simulink model "fw_implement_aux"  (R2026b)
settings: Solver=VariableStepAuto
undefined symbols (not defined in the file or in its folder): ImplementType, P, ShaddadMode, Ts
libraries: simulink x38
settings Model: Creator=aomar  LastModifiedBy=aomar

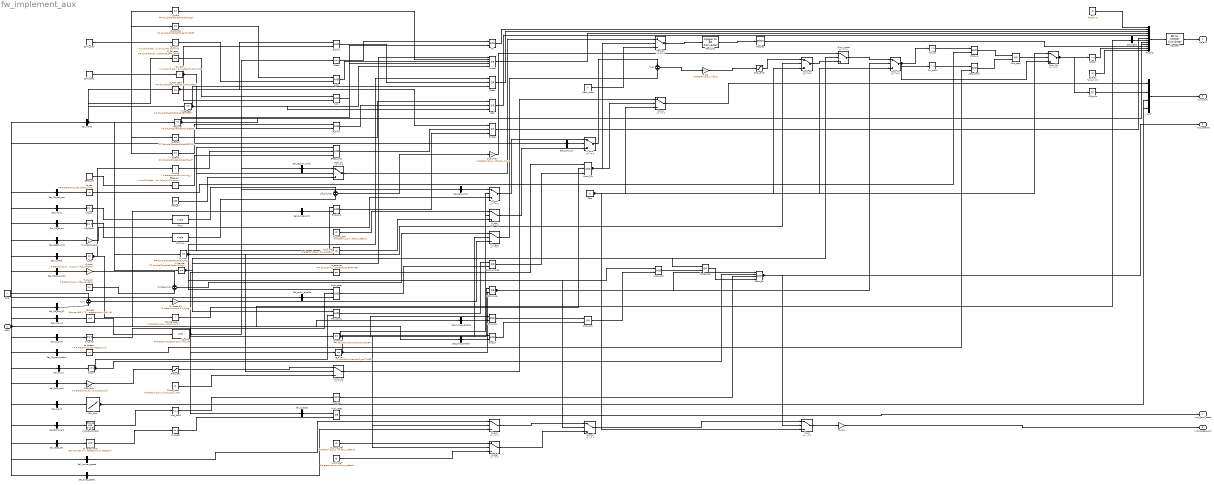
== system fw_implement_aux ==
  fw50 : Inport  SampleTime=Ts.comm
  A_cs : Logic  AllPortsSameDT=off  OutDataTypeStr=boolean
  A_sb : Logic  AllPortsSameDT=off  OutDataTypeStr=boolean
  Amber : Logic  Operator=OR  Inputs=5  AllPortsSameDT=off  OutDataTypeStr=boolean
  At_bottom : simulink/Logic and Bit Operations/Compare To Constant  relop=<=  const=P.electronics.adc.liftpot_lim(1)  OutDataTypeStr=boolean
  At_top : simulink/Logic and Bit Operations/Compare To Constant  relop=>=  const=P.electronics.adc.liftpot_lim(2)  OutDataTypeStr=boolean
  Auto_rotor : Logic  AllPortsSameDT=off  OutDataTypeStr=boolean
  Auto_spray : Logic  Inputs=3  AllPortsSameDT=off  OutDataTypeStr=boolean
  B01 : Constant  Value=false(1,2)  OutDataTypeStr=boolean  SampleTime=Ts.comm
  B19_31 : Constant  Value=false(1,13)  OutDataTypeStr=boolean  SampleTime=Ts.comm
  Beep_auto : Logic  Inputs=3  AllPortsSameDT=off  OutDataTypeStr=boolean
  Beep_cnt : simulink/Sources/Counter Limited  uplimit=round(P.electronics.aux.buzz_period/Ts.comm) - 1  tsamp=Ts.comm
  Beep_on : simulink/Logic and Bit Operations/Compare To Constant  relop=<  const=round(P.electronics.aux.buzz_on/Ts.comm)  OutDataTypeStr=boolean
  Blink_fast : simulink/Sources/Counter Limited  uplimit=round(1/(P.electronics.aux.blink_fast*Ts.comm)) - 1  tsamp=Ts.comm
  Blink_slow : simulink/Sources/Counter Limited  uplimit=round(1/(P.electronics.aux.blink_f*Ts.comm)) - 1  tsamp=Ts.comm
  Buzzer : Logic  Operator=OR  Inputs=3  AllPortsSameDT=off  OutDataTypeStr=boolean
  Di_reset : simulink/Logic and Bit Operations/Compare To Zero  relop=~=  OutDataTypeStr=boolean
  Di_reset_mask : simulink/Logic and Bit Operations/Bitwise Operator  logicop=AND  UseBitMask=on  BitMask=2^(P.electronics.di.reset_btn)  BitMaskRealWorld=Stored Integer
  Dir_down : simulink/Logic and Bit Operations/Compare To Zero  relop=<  OutDataTypeStr=boolean
  Dir_up : simulink/Logic and Bit Operations/Compare To Zero  relop=>  OutDataTypeStr=boolean
  Do_bits : Concatenate  NumInputs=12
  Do_pack : simulink/Logic and Bit Operations/Bit to Integer Converter  nbits=32  bitOrder=LSB first  signedOutputValues=Unsigned  outDtype=uint32  outDtypeSigned=Inherit via internal rule
      settings: LibrarySourceBlock=|
      | commutil2/Bit to Integer
      | Converter
  Down_s : DataTypeConversion  OutDataTypeStr=single  RndMeth=Round
  Duty_a0 : Switch  Criteria=u2 ~= 0  SaturateOnIntegerOverflow=off  InputSameDT=off
  Duty_auto : Saturate  UpperLimit=P.electronics.aux.lift_duty_max  LowerLimit=-P.electronics.aux.lift_duty_max
  Duty_fit : Switch  Criteria=u2 ~= 0  SaturateOnIntegerOverflow=off  InputSameDT=off
  Duty_lift : Switch  Criteria=u2 ~= 0  SaturateOnIntegerOverflow=off  InputSameDT=off
  Duty_man : Gain  Gain=P.electronics.aux.lift_duty_max
  Duty_mode : Switch  Criteria=u2 ~= 0  SaturateOnIntegerOverflow=off  InputSameDT=off
  End_stop : Logic  Operator=OR  AllPortsSameDT=off  OutDataTypeStr=boolean
  Fan_duty : Lookup_n-D  NumberOfTableDimensions=1  BreakpointsForDimension1=P.electronics.aux.fan_bp  BreakpointsForDimension1DataTypeStr=single  Table=P.electronics.aux.fan_duty  TableDataTypeStr=single  ExtrapMethod=Clip  InternalRulePriority=Speed  OutDataTypeStr=single  RndMeth=Simplest
  Fitted : simulink/Logic and Bit Operations/Compare To Constant  relop=~=  const=0  OutDataTypeStr=boolean
  Flow_duty : Gain  Gain=1/P.electronics.aux.pump_flow_full
  Flow_sat : Saturate  UpperLimit=1  LowerLimit=0
  G_blink : Logic  AllPortsSameDT=off  OutDataTypeStr=boolean
  Gnc_buzz : Logic  AllPortsSameDT=off  OutDataTypeStr=boolean
  Gnc_mow : Logic  AllPortsSameDT=off  OutDataTypeStr=boolean
  Gnc_rotor : Logic  Operator=OR  AllPortsSameDT=off  OutDataTypeStr=boolean
  Gnc_till : Logic  AllPortsSameDT=off  OutDataTypeStr=boolean
  Green : Logic  Operator=OR  Inputs=3  AllPortsSameDT=off  OutDataTypeStr=boolean
  H_Kp : Gain  Gain=P.electronics.aux.lift_Kp
  H_cmd : Switch  Criteria=u2 ~= 0  SaturateOnIntegerOverflow=off  InputSameDT=off
  H_cmd_till_gnc : Gain  Gain=-1
  H_def : Switch  Criteria=u2 ~= 0  SaturateOnIntegerOverflow=off  InputSameDT=off
  H_err : Sum  Inputs=+-
  H_gnc : Switch  Criteria=u2 ~= 0  SaturateOnIntegerOverflow=off  InputSameDT=off
  H_meas : Switch  Criteria=u2 ~= 0  SaturateOnIntegerOverflow=off  InputSameDT=off
  H_meas_mow : Sum
  H_meas_till : Gain  Gain=-P.electronics.aux.till_d_max
  H_mow : Gain  Gain=P.electronics.aux.lift_h_range(2) - P.electronics.aux.lift_h_range(1)
  H_mow0 : Constant  Value=P.electronics.aux.lift_h_range(1)  OutDataTypeStr=single  SampleTime=Ts.comm
  H_mow_def : Constant  Value=P.electronics.aux.deck_h_default  OutDataTypeStr=single  SampleTime=Ts.comm
  H_till_def : Constant  Value=-P.electronics.aux.till_d_default  OutDataTypeStr=single  SampleTime=Ts.comm
  Id_mask : simulink/Logic and Bit Operations/Bitwise Operator  logicop=AND  UseBitMask=on  BitMask=2^P.electronics.di.impl_id0 + 2^P.electronics.di.impl_id1  BitMaskRealWorld=Stored Integer
  Id_shift : ArithShift  BitShiftNumber=P.electronics.di.impl_id0  BitShiftDirection=Right
  Impl_fault : simulink/Logic and Bit Operations/Compare To Zero  relop=~=  OutDataTypeStr=boolean
  Impl_fault_mask : simulink/Logic and Bit Operations/Bitwise Operator  logicop=AND  UseBitMask=on  BitMask=2^(28)  BitMaskRealWorld=Stored Integer
  Impl_ok : Logic  Operator=NOT  Inputs=1  AllPortsSameDT=off  OutDataTypeStr=boolean
  Impl_reset : Logic  Operator=OR  AllPortsSameDT=off  OutDataTypeStr=boolean
  Is_mower : simulink/Logic and Bit Operations/Compare To Constant  relop===  const=double(ImplementType.MOWER)  OutDataTypeStr=boolean
  Is_sprayer : simulink/Logic and Bit Operations/Compare To Constant  relop===  const=double(ImplementType.SPRAYER)  OutDataTypeStr=boolean
  Is_tiller : simulink/Logic and Bit Operations/Compare To Constant  relop===  const=double(ImplementType.TILLER)  OutDataTypeStr=boolean
  K3 : Logic  AllPortsSameDT=off  OutDataTypeStr=boolean
  Lift_dir : simulink/Logic and Bit Operations/Compare To Zero  relop=<  OutDataTypeStr=boolean
  Lift_dir_man : Sum  Inputs=+-
  Lift_down : simulink/Logic and Bit Operations/Compare To Constant  relop===  const=3  OutDataTypeStr=boolean
  Lift_pwm : Abs  SaturateOnIntegerOverflow=off
  Lift_up : simulink/Logic and Bit Operations/Compare To Constant  relop===  const=1  OutDataTypeStr=boolean
  M_Auto : simulink/Logic and Bit Operations/Compare To Constant  relop===  const=double(ShaddadMode.AUTO)  OutDataTypeStr=boolean
  M_Auto_start : simulink/Logic and Bit Operations/Compare To Constant  relop===  const=double(ShaddadMode.AUTO_START)  OutDataTypeStr=boolean
  M_Ctrl_stop : simulink/Logic and Bit Operations/Compare To Constant  relop===  const=double(ShaddadMode.CTRL_STOP)  OutDataTypeStr=boolean
  M_Estop : simulink/Logic and Bit Operations/Compare To Constant  relop===  const=double(ShaddadMode.ESTOP)  OutDataTypeStr=boolean
  M_Fault : simulink/Logic and Bit Operations/Compare To Constant  relop===  const=double(ShaddadMode.FAULT)  OutDataTypeStr=boolean
  M_Hold : simulink/Logic and Bit Operations/Compare To Constant  relop===  const=double(ShaddadMode.HOLD)  OutDataTypeStr=boolean
  M_Manual : simulink/Logic and Bit Operations/Compare To Constant  relop===  const=double(ShaddadMode.MANUAL)  OutDataTypeStr=boolean
  M_Selftest : simulink/Logic and Bit Operations/Compare To Constant  relop===  const=double(ShaddadMode.SELFTEST)  OutDataTypeStr=boolean
  M_Standby : simulink/Logic and Bit Operations/Compare To Constant  relop===  const=double(ShaddadMode.STANDBY)  OutDataTypeStr=boolean
  Man_spray : Logic  AllPortsSameDT=off  OutDataTypeStr=boolean
  Mask_all : Constant  Value=255  OutDataTypeStr=uint16  SampleTime=Ts.comm
  Mask_bits : simulink/Logic and Bit Operations/Integer to Bit Converter  nbits=16  signedInputValues=Unsigned  bitOrder=LSB first  outDtype=boolean
      settings: LibrarySourceBlock=|
      | commutil2/Integer to Bit
      | Converter
  Mask_none : Constant  Value=0  OutDataTypeStr=uint16  SampleTime=Ts.comm
  Mask_on : Switch  Criteria=u2 ~= 0  SaturateOnIntegerOverflow=off  InputSameDT=off
  Mask_src : Switch  Criteria=u2 ~= 0  SaturateOnIntegerOverflow=off  InputSameDT=off
  Mode_rotor : Logic  Operator=OR  AllPortsSameDT=off  OutDataTypeStr=boolean
  Moving : simulink/Logic and Bit Operations/Compare To Constant  relop=>  const=P.electronics.aux.moving_v  OutDataTypeStr=boolean
  Moving_spray : simulink/Logic and Bit Operations/Compare To Constant  relop=>  const=P.electronics.aux.spray_v_min  OutDataTypeStr=boolean
  Not_boot : simulink/Logic and Bit Operations/Compare To Constant  relop=~=  const=double(ShaddadMode.BOOT)  OutDataTypeStr=boolean
  Nozzles : Selector  InputPortWidth=16  IndexOptions=Index vector (dialog)  Indices=1:8  OutputSizes=1
  On_fast : simulink/Logic and Bit Operations/Compare To Constant  relop=<  const=round(1/(P.electronics.aux.blink_fast*Ts.comm))/2  OutDataTypeStr=boolean
  On_slow : simulink/Logic and Bit Operations/Compare To Constant  relop=<  const=round(1/(P.electronics.aux.blink_f*Ts.comm))/2  OutDataTypeStr=boolean
  One : Constant  OutDataTypeStr=single  SampleTime=Ts.comm
  Pump : Switch  Criteria=u2 ~= 0  SaturateOnIntegerOverflow=off  InputSameDT=off
  Pump_man : Constant  Value=P.electronics.aux.pump_duty_man  OutDataTypeStr=single  SampleTime=Ts.comm
  Pump_src : Switch  Criteria=u2 ~= 0  SaturateOnIntegerOverflow=off  InputSameDT=off
  Pwm : Concatenate  NumInputs=4
  R_blink : Logic  AllPortsSameDT=off  OutDataTypeStr=boolean
  Red : Logic  Operator=OR  Inputs=3  AllPortsSameDT=off  OutDataTypeStr=boolean
  Rotor_en : Logic  Inputs=4  AllPortsSameDT=off  OutDataTypeStr=boolean
  Rotor_type : Logic  Operator=OR  AllPortsSameDT=off  OutDataTypeStr=boolean
  Sel_T_encl : BusSelector  OutputSignals=adc.T_encl
  Sel_buzzer_cmd : BusSelector  OutputSignals=gnc_cmd.buzzer_cmd
  Sel_comp_ok : BusSelector  OutputSignals=comp_ok
  Sel_deck_cmd : BusSelector  OutputSignals=gnc_cmd.deck_height_cmd
  Sel_depth_cmd : BusSelector  OutputSignals=gnc_cmd.tiller_depth_cmd
  Sel_fault_word : BusSelector  OutputSignals=st.fault_word
  Sel_flow_cmd : BusSelector  OutputSignals=gnc_cmd.spray_flow_cmd
  Sel_impl_id : BusSelector  OutputSignals=di_word
  Sel_lift_down : BusSelector  OutputSignals=st.rc.sw_lift
  Sel_lift_pos_bottom : BusSelector  OutputSignals=adc.lift_pos
  Sel_lift_pos_mow : BusSelector  OutputSignals=adc.lift_pos
  Sel_lift_pos_till : BusSelector  OutputSignals=adc.lift_pos
  Sel_lift_pos_top : BusSelector  OutputSignals=adc.lift_pos
  Sel_lift_up : BusSelector  OutputSignals=st.rc.sw_lift
  Sel_lights : BusSelector  OutputSignals=st.rc.lights
  Sel_mode : BusSelector  OutputSignals=st.mode
  Sel_mower_enable : BusSelector  OutputSignals=gnc_cmd.mower_enable
  Sel_mower_speed : BusSelector  OutputSignals=gnc_cmd.mower_speed_cmd
  Sel_rc_reset : BusSelector  OutputSignals=st.rc.reset_req
  Sel_reset_btn : BusSelector  OutputSignals=di_word
  Sel_section_mask : BusSelector  OutputSignals=gnc_cmd.spray_section_mask
  Sel_spray_enable : BusSelector  OutputSignals=gnc_cmd.spray_enable
  Sel_sw_auto : BusSelector  OutputSignals=st.rc.sw_impl
  Sel_sw_on : BusSelector  OutputSignals=st.rc.sw_impl
  Sel_tiller_enable : BusSelector  OutputSignals=gnc_cmd.tiller_enable
  Sel_tiller_speed : BusSelector  OutputSignals=gnc_cmd.tiller_speed_cmd
  Sel_v_track : BusSelector  OutputSignals=st.v_track
  Spray_mode : Logic  Operator=OR  AllPortsSameDT=off  OutDataTypeStr=boolean
  Spray_on : Logic  Inputs=3  AllPortsSameDT=off  OutDataTypeStr=boolean
  Stop_down : Logic  AllPortsSameDT=off  OutDataTypeStr=boolean
  Stop_up : Logic  AllPortsSameDT=off  OutDataTypeStr=boolean
  Sw_auto : simulink/Logic and Bit Operations/Compare To Constant  relop===  const=3  OutDataTypeStr=boolean
  Sw_on : simulink/Logic and Bit Operations/Compare To Constant  relop=>=  const=2  OutDataTypeStr=boolean
  To_rpm : Gain  Gain=30/pi
  Up_s : DataTypeConversion  OutDataTypeStr=single  RndMeth=Round
  V_abs : Abs  SaturateOnIntegerOverflow=off
  W_cmd : Switch  Criteria=u2 ~= 0  SaturateOnIntegerOverflow=off  InputSameDT=off
  W_def : Switch  Criteria=u2 ~= 0  SaturateOnIntegerOverflow=off  InputSameDT=off
  W_gnc : Switch  Criteria=u2 ~= 0  SaturateOnIntegerOverflow=off  InputSameDT=off
  W_mow_def : Constant  Value=P.electronics.aux.mower_w_default  OutDataTypeStr=single  SampleTime=Ts.comm
  W_on : Switch  Criteria=u2 ~= 0  SaturateOnIntegerOverflow=off  InputSameDT=off
  W_till_def : Constant  Value=P.electronics.aux.tiller_w_default  OutDataTypeStr=single  SampleTime=Ts.comm
  X_inv : Sum  Inputs=+-
  Zero : Constant  Value=0  OutDataTypeStr=single  SampleTime=Ts.comm
  do_aux : Outport  OutDataTypeStr=uint32
  pwm_duty : Outport  Port=2  OutDataTypeStr=single
  impl_enable : Outport  Port=3  OutDataTypeStr=boolean
  impl_fault_reset : Outport  Port=4  OutDataTypeStr=boolean
  impl_speed_rpm : Outport  Port=5  OutDataTypeStr=single
  wires:
  One/1 -> X_inv/1  "One"
  fw50/1 -> Sel_lights/1, Sel_mode/1, Sel_comp_ok/1, Sel_section_mask/1, Sel_tiller_speed/1, Sel_deck_cmd/1, Sel_lift_pos_top/1, Sel_mower_speed/1, Sel_lift_up/1, Sel_reset_btn/1, Sel_buzzer_cmd/1, Sel_lift_down/1, Sel_fault_word/1, Sel_depth_cmd/1, Sel_rc_reset/1, Sel_T_encl/1, Sel_v_track/1, Sel_flow_cmd/1, Sel_lift_pos_mow/1, Sel_sw_on/1, Sel_spray_enable/1, Sel_lift_pos_bottom/1, Sel_lift_pos_till/1, Sel_tiller_enable/1, Sel_sw_auto/1, Sel_impl_id/1, Sel_mower_enable/1  "fw50"
  Sel_lift_pos_top/1 -> At_top/1  "<lift_pos>"
  Sel_lift_up/1 -> Lift_up/1  "<sw_lift>"
  Sel_lift_down/1 -> Lift_down/1  "<sw_lift>"
  Sel_depth_cmd/1 -> H_cmd_till_gnc/1  "<tiller_depth_cmd>"
  Sel_v_track/1 -> V_abs/1  "<v_track>"
  Sel_lift_pos_mow/1 -> H_mow/1  "<lift_pos>"
  Sel_lift_pos_till/1 -> X_inv/2  "<lift_pos>"
  Sel_impl_id/1 -> Id_mask/1  "<di_word>"
  Sel_sw_auto/1 -> Sw_auto/1  "<sw_impl>"
  Sel_lift_pos_bottom/1 -> At_bottom/1  "<lift_pos>"
  Sel_flow_cmd/1 -> Flow_duty/1  "<spray_flow_cmd>"
  Sel_T_encl/1 -> Fan_duty/1  "<T_encl>"
  Sel_fault_word/1 -> Impl_fault_mask/1  "<fault_word>"
  Sel_reset_btn/1 -> Di_reset_mask/1  "<di_word>"
  Sel_sw_on/1 -> Sw_on/1  "<sw_impl>"
  Sel_mode/1 -> M_Manual/1, M_Auto/1, M_Hold/1, M_Standby/1, M_Ctrl_stop/1, M_Auto_start/1, M_Fault/1, M_Estop/1, M_Selftest/1, Not_boot/1  "<mode>"
  Sel_mower_speed/1 -> W_gnc/1  "<mower_speed_cmd>"
  Sel_tiller_speed/1 -> W_gnc/3  "<tiller_speed_cmd>"
  X_inv/1 -> H_meas_till/1  "X_inv"
  Blink_slow/1 -> On_slow/1  "Blink_slow"
  Blink_fast/1 -> On_fast/1  "Blink_fast"
  Beep_cnt/1 -> Beep_on/1  "Beep_cnt"
  At_top/1 -> Stop_up/2  "At_top"
  Lift_up/1 -> Up_s/1  "Lift_up"
  Lift_down/1 -> Down_s/1  "Lift_down"
  H_cmd_till_gnc/1 -> H_gnc/3  "H_cmd_till_gnc"
  V_abs/1 -> Moving/1, Moving_spray/1  "V_abs"
  H_mow/1 -> H_meas_mow/1  "H_mow"
  H_mow0/1 -> H_meas_mow/2  "H_mow0"
  Sw_auto/1 -> Auto_spray/2  "Sw_auto"
  At_bottom/1 -> Stop_down/2  "At_bottom"
  Flow_duty/1 -> Flow_sat/1  "Flow_duty"
  Id_mask/1 -> Id_shift/1  "Id_mask"
  Sw_on/1 -> Rotor_en/2, Man_spray/2  "Sw_on"
  Impl_fault_mask/1 -> Impl_fault/1  "Impl_fault_mask"
  Di_reset_mask/1 -> Di_reset/1  "Di_reset_mask"
  Fan_duty/1 -> Pwm/3, Pwm/4  "fan_duty"
  H_meas_mow/1 -> H_meas/1  "H_meas_mow"
  M_Hold/1 -> Amber/2  "M_Hold"
  M_Standby/1 -> A_sb/1  "M_Standby"
  On_slow/1 -> A_sb/2  "On_slow"
  M_Ctrl_stop/1 -> A_cs/1  "M_Ctrl_stop"
  M_Auto_start/1 -> G_blink/1, Buzzer/1  "M_Auto_start"
  M_Estop/1 -> Red/1  "M_Estop"
  M_Fault/1 -> R_blink/1  "M_Fault"
  Moving/1 -> Beep_auto/2  "Moving"
  Beep_on/1 -> Beep_auto/3  "Beep_on"
  Mask_all/1 -> Mask_src/3  "Mask_all"
  H_meas_till/1 -> H_meas/3  "H_meas_till"
  Moving_spray/1 -> Spray_on/2  "Moving_spray"
  Flow_sat/1 -> Pump_src/1  "Flow_sat"
  Pump_man/1 -> Pump_src/3  "Pump_man"
  Impl_fault/1 -> Impl_ok/1  "impl_fault"
  Di_reset/1 -> Impl_reset/2  "Di_reset"
  Not_boot/1 -> Do_bits/8, Do_bits/9, K3/2  "Not_boot"
  On_fast/1 -> R_blink/2, G_blink/2, A_cs/2  "On_fast"
  M_Manual/1 -> Amber/1, Duty_mode/2, Man_spray/1, Mode_rotor/1  "M_Manual"
  M_Auto/1 -> Duty_a0/2, Green/1, W_cmd/2, Pump_src/2, Beep_auto/1, Mask_src/2, Gnc_buzz/1, Auto_spray/1, Auto_rotor/1  "M_Auto"
  Up_s/1 -> Lift_dir_man/1  "Up_s"
  Down_s/1 -> Lift_dir_man/2  "Down_s"
  Id_shift/1 -> Fitted/1, Is_sprayer/1, Is_tiller/1, Is_mower/1  "impl_id"
  M_Selftest/1 -> Amber/5, Green/3, Red/3  "M_Selftest"
  Sel_section_mask/1 -> Mask_src/1  "<spray_section_mask>"
  Sel_buzzer_cmd/1 -> Gnc_buzz/2  "<buzzer_cmd>"
  Sel_spray_enable/1 -> Auto_spray/3  "<spray_enable>"
  Sel_rc_reset/1 -> Impl_reset/1  "<reset_req>"
  Lift_dir_man/1 -> Duty_man/1  "Lift_dir_man"
  G_blink/1 -> Green/2  "G_blink"
  Fitted/1 -> K3/1  "Fitted"
  A_sb/1 -> Amber/3  "A_sb"
  A_cs/1 -> Amber/4  "A_cs"
  R_blink/1 -> Red/2  "R_blink"
  Beep_auto/1 -> Buzzer/2  "Beep_auto"
  Gnc_buzz/1 -> Buzzer/3  "Gnc_buzz"
  H_mow_def/1 -> H_def/1  "H_mow_def"
  H_till_def/1 -> H_def/3  "H_till_def"
  Is_sprayer/1 -> Spray_on/1  "Is_sprayer"
  Auto_spray/1 -> Spray_mode/2  "Auto_spray"
  Man_spray/1 -> Spray_mode/1  "Man_spray"
  Is_mower/1 -> H_gnc/2, H_def/2, W_def/2, H_meas/2, W_gnc/2, Rotor_type/1, Gnc_mow/1  "Is_mower"
  Impl_ok/1 -> Rotor_en/3  "Impl_ok"
  Impl_reset/1 -> impl_fault_reset/1  "impl_fault_reset"
  W_mow_def/1 -> W_def/1  "W_mow_def"
  W_till_def/1 -> W_def/3  "W_till_def"
  Is_tiller/1 -> Rotor_type/2, Gnc_till/1  "Is_tiller"
  Mask_src/1 -> Mask_on/1  "Mask_src"
  Pump_src/1 -> Pump/1  "Pump_src"
  Sel_deck_cmd/1 -> H_gnc/1  "<deck_height_cmd>"
  Sel_mower_enable/1 -> Gnc_mow/2  "<mower_enable>"
  Sel_tiller_enable/1 -> Gnc_till/2  "<tiller_enable>"
  K3/1 -> Do_bits/2  "K3"
  Amber/1 -> Do_bits/4  "Amber"
  Green/1 -> Do_bits/3  "Green"
  Red/1 -> Do_bits/5  "Red"
  Buzzer/1 -> Do_bits/6  "Buzzer"
  Duty_man/1 -> Duty_mode/1  "Duty_man"
  Spray_mode/1 -> Spray_on/3  "Spray_mode"
  Rotor_type/1 -> Duty_fit/2, Rotor_en/1  "Rotor_type"
  Gnc_mow/1 -> Gnc_rotor/1  "Gnc_mow"
  Gnc_till/1 -> Gnc_rotor/2  "Gnc_till"
  H_gnc/1 -> H_cmd/1  "H_gnc"
  H_def/1 -> H_cmd/3  "H_def"
  H_meas/1 -> H_err/2  "h_meas"
  W_gnc/1 -> W_cmd/1  "W_gnc"
  W_def/1 -> W_cmd/3  "W_def"
  Sel_comp_ok/1 -> H_cmd/2  "<comp_ok>"
  Mask_none/1 -> Mask_on/3  "Mask_none"
  Spray_on/1 -> Mask_on/2, Pump/2  "spray_on"
  Gnc_rotor/1 -> Auto_rotor/2  "Gnc_rotor"
  Zero/1 -> W_on/3, Duty_lift/1, Duty_a0/3, Duty_fit/3, Pump/3  "Zero"
  H_cmd/1 -> H_err/1  "h_cmd"
  W_cmd/1 -> W_on/1  "w_impl"
  H_err/1 -> H_Kp/1  "H_err"
  Auto_rotor/1 -> Mode_rotor/2  "Auto_rotor"
  Mask_on/1 -> Mask_bits/1  "nozzle_mask"
  Pump/1 -> Pwm/1  "pump_duty"
  H_Kp/1 -> Duty_auto/1  "H_Kp"
  Mode_rotor/1 -> Rotor_en/4  "Mode_rotor"
  Mask_bits/1 -> Nozzles/1  "Mask_bits"
  Duty_auto/1 -> Duty_a0/1  "Duty_auto"
  Rotor_en/1 -> impl_enable/1, W_on/2  "rotor_en"
  Nozzles/1 -> Do_bits/10  "Nozzles"
  Duty_a0/1 -> Duty_mode/3  "Duty_a0"
  W_on/1 -> To_rpm/1  "W_on"
  To_rpm/1 -> impl_speed_rpm/1  "impl_speed_rpm"
  Duty_mode/1 -> Duty_fit/1  "lift_duty_req"
  Duty_fit/1 -> Dir_up/1, Dir_down/1, Duty_lift/3  "Duty_fit"
  Dir_up/1 -> Stop_up/1  "Dir_up"
  Dir_down/1 -> Stop_down/1  "Dir_down"
  Stop_up/1 -> End_stop/1  "Stop_up"
  Stop_down/1 -> End_stop/2  "Stop_down"
  End_stop/1 -> Duty_lift/2  "end_stop"
  Duty_lift/1 -> Lift_pwm/1, Lift_dir/1  "lift_duty"
  B01/1 -> Do_bits/1  "B01"
  Lift_dir/1 -> Do_bits/11  "Lift_dir"
  B19_31/1 -> Do_bits/12  "B19_31"
  Lift_pwm/1 -> Pwm/2  "Lift_pwm"
  Sel_lights/1 -> Do_bits/7  "<lights>"
  Do_bits/1 -> Do_pack/1  "do_bits"
  Pwm/1 -> pwm_duty/1  "pwm_duty"
  Do_pack/1 -> do_aux/1  "do_aux"
